simulink model "balance_car_measured_foc"  (R2025b)
settings: Solver=ode15s  StartTime=0.0  StopTime=6  MaxStep=0.00025  RelTol=1e-5  AbsTol=1e-7
PostLoadFcn:
  | addpath(fileparts(get_param(bdroot,'FileName')));addpath(fileparts(fileparts(get_param(bdroot,'FileName'))));p=balance_setup;addpath(fullfile(p.root,'模型','仿真模型','通用URDF','meshes'));
model workspace (MAT data in the model file):
  direction_convention = 'x_right_y_forward_v2'
  foc_config = [0.110387231165 2.4e-05 0.00887463966788 0.060318579 226.194672 5e-05 4 3 8.03 0.04 0.4 0.7 ... (31 elements, 1x31)]
  sensor_config = [1 0.314910266476 0.419379363666 0.000198810278564 0.000166561121409 0.00015843402401 0.005 44 0.0325 0.00147678407027 4.07299587781e-05 1.77121446999e-05 ... (342 elements, 1x342)]
  suite_config = [1 0.7 -0.00156420808869 0 0 0 0 0 0 0 0 0 ... (37 elements, 1x37)]
  terrain_dimensions = [0.3  0.120037494142  0.01; 0.3  0.1  0.01; 0.3  0.120037494142  0.01; 0.06  0.04  0.01]
  terrain_on = 0
  terrain_rotation_deg = [-1.43209618416; 0; 1.43209618416; 0]
  terrain_translation = [0  0.240124960956  -0.00349843823204; 0  0.35  -0.002; 0  0.459875039044  -0.00349843823204; -0.0662682  0.62  -0.0042]
values from neighbouring files (symbols this model uses):
  N = numel(t)    [screen_measured_pid.m]
  s = load(fullfile(folder,'simulation_measured.mat'),'o')    [analyze_course_odometry.m]    (also in build_measured_car.m = side{1}; diagnose_encoder_yaw_gate.m = jsondecode(fileread(fullfile(out,'summary.json'))); measured_car_reference.m = amplitude*(10*u^3-15*u^4+6*u^5); measured_ekf_step.m = [0 -v(3) v(2);v(3) 0 -v(1);-v(2) v(1) 0])
  Y = []    [identify_measured_foc.m]
undefined symbols (not defined in the file or in its folder): X, Z
libraries: sm_lib x48, nesl_utility x27
(part 2 of 2)

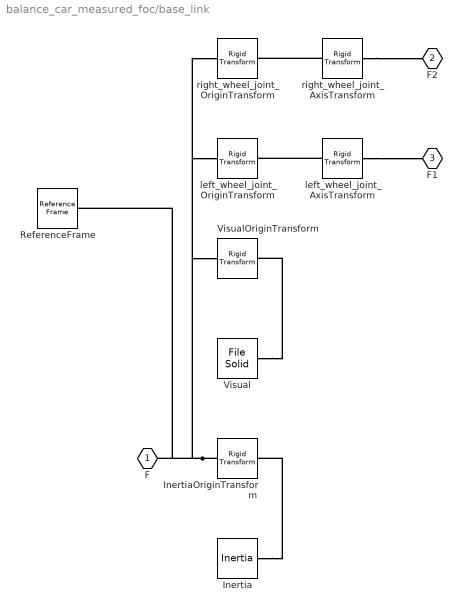
== system balance_car_measured_foc/base_link ==
  Inertia : sm_lib/Body Elements/Inertia  InertiaType=Custom  Mass=0.2771  MassUnits=kg  CenterOfMass=[0, 0, 0]  CenterOfMassUnits=m  MomentsOfInertia=[0.000311847668361045, 0.0006191390109428378, 0.000388176637385571]  MomentsOfInertiaUnits=kg*m^2  ProductsOfInertia=[3.850274462317628e-08, -1.767576624229698e-07, -2.823397326959528e-07]  ProductsOfInertiaUnits=kg*m^2  GraphicType=None  MarkerShape=Inertia  MarkerSize=20  GraphicVisPropType=SimpleVisualProperties  GraphicDiffuseColor=[0.5 0.5 0.5]  GraphicOpacity=1  GraphicSpecularColor=[0.5 0.5 0.5 1.0]  GraphicAmbientColor=[0.15 0.15 0.15 1.0]  GraphicEmissiveColor=[0.0 0.0 0.0 1.0]  GraphicShininess=75
  InertiaOriginTransform : sm_lib/Frames and Transforms/Rigid Transform  RotationMethod=RotationSequence  FollAlignAxisA=+X  BaseAlignAxisA=+Y  FollAlignAxisB=+Y  BaseAlignAxisB=+Z  RotationStandardAxis=+Z  RotationAngle=0  RotationAngleUnits=deg  RotationArbitraryAxis=[0 0 1]  RotationSequenceAxes=BaseAxes  RotationSequence=XYZ  RotationSequenceAngles=[0, 0, 0]  RotationSequenceAnglesUnits=rad  RotationMatrix=[1 0 0;0 1 0;0 0 1]  Quaternion=[1 0 0 0]  TranslationMethod=Cartesian  TranslationCartesianOffset=[-4.53146929236e-05, 5.71393596063e-05, 0.0365292274203]  TranslationCartesianOffsetUnits=m  TranslationStandardAxis=+Z  TranslationStandardOffset=0  TranslationStandardOffsetUnits=m  TranslationROffset=0  TranslationROffsetUnits=m  TranslationThetaOffset=0  TranslationThetaOffsetUnits=deg  TranslationZOffset=0  TranslationZOffsetUnits=m
  ReferenceFrame : sm_lib/Frames and Transforms/Reference Frame
  Visual : sm_lib/Body Elements/File Solid  ExtGeomFileName=body.stl  UnitType=Custom  ExtGeomFileUnits=m  StepReaderType=HEX  ExportConvexHullGeometry=off  InertiaType=Custom  BasedOnType=DensityFromFile  Density=1000  DensityUnits=kg/m^3  Mass=0  MassUnits=kg  CenterOfMass=[0, 0, 0]  CenterOfMassUnits=m  MomentsOfInertia=[0, 0, 0]  MomentsOfInertiaUnits=kg*m^2  ProductsOfInertia=[0, 0, 0]  ProductsOfInertiaUnits=kg*m^2  GraphicType=FromGeometry  MarkerShape=Sphere  MarkerSize=10  GraphicVisPropType=SimpleVisualProperties  GraphicDiffuseColor=[0.12, 0.4, 0.65]  GraphicOpacity=1  GraphicSpecularColor=[0.5 0.5 0.5 1.0]  GraphicAmbientColor=[0.15 0.15 0.15 1.0]  GraphicEmissiveColor=[0.0 0.0 0.0 1.0]  GraphicShininess=75  DoExposeReferenceFrame=on  SerializedFrames=<Frames/>
  VisualOriginTransform : sm_lib/Frames and Transforms/Rigid Transform  RotationMethod=RotationSequence  FollAlignAxisA=+X  BaseAlignAxisA=+Y  FollAlignAxisB=+Y  BaseAlignAxisB=+Z  RotationStandardAxis=+Z  RotationAngle=0  RotationAngleUnits=deg  RotationArbitraryAxis=[0 0 1]  RotationSequenceAxes=BaseAxes  RotationSequence=XYZ  RotationSequenceAngles=[0, 0, -1.570796326794897]  RotationSequenceAnglesUnits=rad  RotationMatrix=[1 0 0;0 1 0;0 0 1]  Quaternion=[1 0 0 0]  TranslationMethod=Cartesian  TranslationCartesianOffset=[0, 0, 0]  TranslationCartesianOffsetUnits=m  TranslationStandardAxis=+Z  TranslationStandardOffset=0  TranslationStandardOffsetUnits=m  TranslationROffset=0  TranslationROffsetUnits=m  TranslationThetaOffset=0  TranslationThetaOffsetUnits=deg  TranslationZOffset=0  TranslationZOffsetUnits=m
  left_wheel_joint_AxisTransform : sm_lib/Frames and Transforms/Rigid Transform  RotationMethod=ArbitraryAxis  FollAlignAxisA=+X  BaseAlignAxisA=+Y  FollAlignAxisB=+Y  BaseAlignAxisB=+Z  RotationStandardAxis=+Z  RotationAngle=1.570796326794897  RotationAngleUnits=rad  RotationArbitraryAxis=[-0, -1, 0]  RotationSequenceAxes=FollowerAxes  RotationSequence=XYX  RotationSequenceAngles=[0 0 0]  RotationSequenceAnglesUnits=deg  RotationMatrix=[1 0 0;0 1 0;0 0 1]  Quaternion=[1 0 0 0]  TranslationMethod=Cartesian  TranslationCartesianOffset=[0, 0, 0]  TranslationCartesianOffsetUnits=m  TranslationStandardAxis=+Z  TranslationStandardOffset=0  TranslationStandardOffsetUnits=m  TranslationROffset=0  TranslationROffsetUnits=m  TranslationThetaOffset=0  TranslationThetaOffsetUnits=deg  TranslationZOffset=0  TranslationZOffsetUnits=m
  left_wheel_joint_OriginTransform : sm_lib/Frames and Transforms/Rigid Transform  RotationMethod=RotationSequence  FollAlignAxisA=+X  BaseAlignAxisA=+Y  FollAlignAxisB=+Y  BaseAlignAxisB=+Z  RotationStandardAxis=+Z  RotationAngle=0  RotationAngleUnits=deg  RotationArbitraryAxis=[0 0 1]  RotationSequenceAxes=BaseAxes  RotationSequence=XYZ  RotationSequenceAngles=[0, 0, 0]  RotationSequenceAnglesUnits=rad  RotationMatrix=[1 0 0;0 1 0;0 0 1]  Quaternion=[1 0 0 0]  TranslationMethod=Cartesian  TranslationCartesianOffset=[-0.0662682, 0, 0]  TranslationCartesianOffsetUnits=m  TranslationStandardAxis=+Z  TranslationStandardOffset=0  TranslationStandardOffsetUnits=m  TranslationROffset=0  TranslationROffsetUnits=m  TranslationThetaOffset=0  TranslationThetaOffsetUnits=deg  TranslationZOffset=0  TranslationZOffsetUnits=m
  right_wheel_joint_AxisTransform : sm_lib/Frames and Transforms/Rigid Transform  RotationMethod=ArbitraryAxis  FollAlignAxisA=+X  BaseAlignAxisA=+Y  FollAlignAxisB=+Y  BaseAlignAxisB=+Z  RotationStandardAxis=+Z  RotationAngle=1.570796326794897  RotationAngleUnits=rad  RotationArbitraryAxis=[-0, -1, 0]  RotationSequenceAxes=FollowerAxes  RotationSequence=XYX  RotationSequenceAngles=[0 0 0]  RotationSequenceAnglesUnits=deg  RotationMatrix=[1 0 0;0 1 0;0 0 1]  Quaternion=[1 0 0 0]  TranslationMethod=Cartesian  TranslationCartesianOffset=[0, 0, 0]  TranslationCartesianOffsetUnits=m  TranslationStandardAxis=+Z  TranslationStandardOffset=0  TranslationStandardOffsetUnits=m  TranslationROffset=0  TranslationROffsetUnits=m  TranslationThetaOffset=0  TranslationThetaOffsetUnits=deg  TranslationZOffset=0  TranslationZOffsetUnits=m
  right_wheel_joint_OriginTransform : sm_lib/Frames and Transforms/Rigid Transform  RotationMethod=RotationSequence  FollAlignAxisA=+X  BaseAlignAxisA=+Y  FollAlignAxisB=+Y  BaseAlignAxisB=+Z  RotationStandardAxis=+Z  RotationAngle=0  RotationAngleUnits=deg  RotationArbitraryAxis=[0 0 1]  RotationSequenceAxes=BaseAxes  RotationSequence=XYZ  RotationSequenceAngles=[0, 0, 0]  RotationSequenceAnglesUnits=rad  RotationMatrix=[1 0 0;0 1 0;0 0 1]  Quaternion=[1 0 0 0]  TranslationMethod=Cartesian  TranslationCartesianOffset=[0.0662682, 0, 0]  TranslationCartesianOffsetUnits=m  TranslationStandardAxis=+Z  TranslationStandardOffset=0  TranslationStandardOffsetUnits=m  TranslationROffset=0  TranslationROffsetUnits=m  TranslationThetaOffset=0  TranslationThetaOffsetUnits=deg  TranslationZOffset=0  TranslationZOffsetUnits=m
  F : PMIOPort  Side=Left
  F2 : PMIOPort  Port=2  Side=Right
  F1 : PMIOPort  Port=3  Side=Right
  connections:
  Inertia/RConn1 -- InertiaOriginTransform/RConn1
  ReferenceFrame/RConn1 -- InertiaOriginTransform/LConn1 -- VisualOriginTransform/LConn1 -- left_wheel_joint_OriginTransform/LConn1 -- right_wheel_joint_OriginTransform/LConn1 -- F/RConn1
  Visual/RConn1 -- VisualOriginTransform/RConn1
  left_wheel_joint_AxisTransform/RConn1 -- F1/RConn1
  left_wheel_joint_AxisTransform/LConn1 -- left_wheel_joint_OriginTransform/RConn1
  right_wheel_joint_AxisTransform/RConn1 -- F2/RConn1
  right_wheel_joint_AxisTransform/LConn1 -- right_wheel_joint_OriginTransform/RConn1

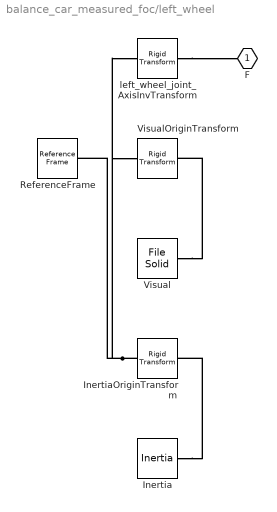
== system balance_car_measured_foc/left_wheel ==
  Inertia : sm_lib/Body Elements/Inertia  InertiaType=Custom  Mass=0.06270000000000001  MassUnits=kg  CenterOfMass=[0, 0, 0]  CenterOfMassUnits=m  MomentsOfInertia=[2.996788998409583e-05, 1.917831991019923e-05, 1.917831830082714e-05]  MomentsOfInertiaUnits=kg*m^2  ProductsOfInertia=[-7.252640957165455e-12, -1.265848447928984e-12, -3.833693155565584e-12]  ProductsOfInertiaUnits=kg*m^2  GraphicType=None  MarkerShape=Inertia  MarkerSize=20  GraphicVisPropType=SimpleVisualProperties  GraphicDiffuseColor=[0.5 0.5 0.5]  GraphicOpacity=1  GraphicSpecularColor=[0.5 0.5 0.5 1.0]  GraphicAmbientColor=[0.15 0.15 0.15 1.0]  GraphicEmissiveColor=[0.0 0.0 0.0 1.0]  GraphicShininess=75
  InertiaOriginTransform : sm_lib/Frames and Transforms/Rigid Transform  RotationMethod=RotationSequence  FollAlignAxisA=+X  BaseAlignAxisA=+Y  FollAlignAxisB=+Y  BaseAlignAxisB=+Z  RotationStandardAxis=+Z  RotationAngle=0  RotationAngleUnits=deg  RotationArbitraryAxis=[0 0 1]  RotationSequenceAxes=BaseAxes  RotationSequence=XYZ  RotationSequenceAngles=[0, 0, 0]  RotationSequenceAnglesUnits=rad  RotationMatrix=[1 0 0;0 1 0;0 0 1]  Quaternion=[1 0 0 0]  TranslationMethod=Cartesian  TranslationCartesianOffset=[0.00137780420767, 3.60871449808e-09, -5.37617755869e-09]  TranslationCartesianOffsetUnits=m  TranslationStandardAxis=+Z  TranslationStandardOffset=0  TranslationStandardOffsetUnits=m  TranslationROffset=0  TranslationROffsetUnits=m  TranslationThetaOffset=0  TranslationThetaOffsetUnits=deg  TranslationZOffset=0  TranslationZOffsetUnits=m
  ReferenceFrame : sm_lib/Frames and Transforms/Reference Frame
  Visual : sm_lib/Body Elements/File Solid  ExtGeomFileName=right_wheel.stl  UnitType=Custom  ExtGeomFileUnits=m  StepReaderType=HEX  ExportConvexHullGeometry=off  InertiaType=Custom  BasedOnType=DensityFromFile  Density=1000  DensityUnits=kg/m^3  Mass=0  MassUnits=kg  CenterOfMass=[0, 0, 0]  CenterOfMassUnits=m  MomentsOfInertia=[0, 0, 0]  MomentsOfInertiaUnits=kg*m^2  ProductsOfInertia=[0, 0, 0]  ProductsOfInertiaUnits=kg*m^2  GraphicType=FromGeometry  MarkerShape=Sphere  MarkerSize=10  GraphicVisPropType=SimpleVisualProperties  GraphicDiffuseColor=[0.16, 0.18, 0.16]  GraphicOpacity=1  GraphicSpecularColor=[0.5 0.5 0.5 1.0]  GraphicAmbientColor=[0.15 0.15 0.15 1.0]  GraphicEmissiveColor=[0.0 0.0 0.0 1.0]  GraphicShininess=75  DoExposeReferenceFrame=on  SerializedFrames=<Frames/>
  VisualOriginTransform : sm_lib/Frames and Transforms/Rigid Transform  RotationMethod=RotationSequence  FollAlignAxisA=+X  BaseAlignAxisA=+Y  FollAlignAxisB=+Y  BaseAlignAxisB=+Z  RotationStandardAxis=+Z  RotationAngle=0  RotationAngleUnits=deg  RotationArbitraryAxis=[0 0 1]  RotationSequenceAxes=BaseAxes  RotationSequence=XYZ  RotationSequenceAngles=[0, 0, -1.570796326794897]  RotationSequenceAnglesUnits=rad  RotationMatrix=[1 0 0;0 1 0;0 0 1]  Quaternion=[1 0 0 0]  TranslationMethod=Cartesian  TranslationCartesianOffset=[0, 0, 0]  TranslationCartesianOffsetUnits=m  TranslationStandardAxis=+Z  TranslationStandardOffset=0  TranslationStandardOffsetUnits=m  TranslationROffset=0  TranslationROffsetUnits=m  TranslationThetaOffset=0  TranslationThetaOffsetUnits=deg  TranslationZOffset=0  TranslationZOffsetUnits=m
  left_wheel_joint_AxisInvTransform : sm_lib/Frames and Transforms/Rigid Transform  RotationMethod=ArbitraryAxis  FollAlignAxisA=+X  BaseAlignAxisA=+Y  FollAlignAxisB=+Y  BaseAlignAxisB=+Z  RotationStandardAxis=+Z  RotationAngle=1.570796326794897  RotationAngleUnits=rad  RotationArbitraryAxis=[-0, -1, 0]  RotationSequenceAxes=FollowerAxes  RotationSequence=XYX  RotationSequenceAngles=[0 0 0]  RotationSequenceAnglesUnits=deg  RotationMatrix=[1 0 0;0 1 0;0 0 1]  Quaternion=[1 0 0 0]  TranslationMethod=Cartesian  TranslationCartesianOffset=[0, 0, 0]  TranslationCartesianOffsetUnits=m  TranslationStandardAxis=+Z  TranslationStandardOffset=0  TranslationStandardOffsetUnits=m  TranslationROffset=0  TranslationROffsetUnits=m  TranslationThetaOffset=0  TranslationThetaOffsetUnits=deg  TranslationZOffset=0  TranslationZOffsetUnits=m
  F : PMIOPort  Side=Left
  connections:
  Inertia/RConn1 -- InertiaOriginTransform/RConn1
  ReferenceFrame/RConn1 -- InertiaOriginTransform/LConn1 -- VisualOriginTransform/LConn1 -- left_wheel_joint_AxisInvTransform/LConn1
  Visual/RConn1 -- VisualOriginTransform/RConn1
  left_wheel_joint_AxisInvTransform/RConn1 -- F/RConn1

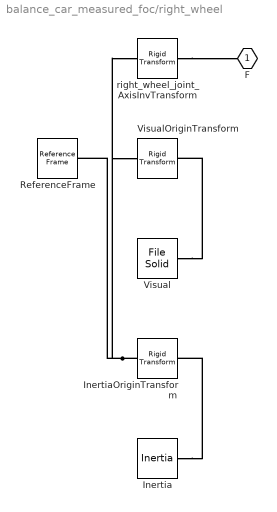
== system balance_car_measured_foc/right_wheel ==
  Inertia : sm_lib/Body Elements/Inertia  InertiaType=Custom  Mass=0.06270000000000001  MassUnits=kg  CenterOfMass=[0, 0, 0]  CenterOfMassUnits=m  MomentsOfInertia=[2.996788998409583e-05, 1.917831991019924e-05, 1.917831830082714e-05]  MomentsOfInertiaUnits=kg*m^2  ProductsOfInertia=[7.252640958073256e-12, 1.265848450812081e-12, -3.83369315636605e-12]  ProductsOfInertiaUnits=kg*m^2  GraphicType=None  MarkerShape=Inertia  MarkerSize=20  GraphicVisPropType=SimpleVisualProperties  GraphicDiffuseColor=[0.5 0.5 0.5]  GraphicOpacity=1  GraphicSpecularColor=[0.5 0.5 0.5 1.0]  GraphicAmbientColor=[0.15 0.15 0.15 1.0]  GraphicEmissiveColor=[0.0 0.0 0.0 1.0]  GraphicShininess=75
  InertiaOriginTransform : sm_lib/Frames and Transforms/Rigid Transform  RotationMethod=RotationSequence  FollAlignAxisA=+X  BaseAlignAxisA=+Y  FollAlignAxisB=+Y  BaseAlignAxisB=+Z  RotationStandardAxis=+Z  RotationAngle=0  RotationAngleUnits=deg  RotationArbitraryAxis=[0 0 1]  RotationSequenceAxes=BaseAxes  RotationSequence=XYZ  RotationSequenceAngles=[0, 0, 0]  RotationSequenceAnglesUnits=rad  RotationMatrix=[1 0 0;0 1 0;0 0 1]  Quaternion=[1 0 0 0]  TranslationMethod=Cartesian  TranslationCartesianOffset=[-0.00137780420767, -3.60871449673e-09, -5.37617755869e-09]  TranslationCartesianOffsetUnits=m  TranslationStandardAxis=+Z  TranslationStandardOffset=0  TranslationStandardOffsetUnits=m  TranslationROffset=0  TranslationROffsetUnits=m  TranslationThetaOffset=0  TranslationThetaOffsetUnits=deg  TranslationZOffset=0  TranslationZOffsetUnits=m
  ReferenceFrame : sm_lib/Frames and Transforms/Reference Frame
  Visual : sm_lib/Body Elements/File Solid  ExtGeomFileName=left_wheel.stl  UnitType=Custom  ExtGeomFileUnits=m  StepReaderType=HEX  ExportConvexHullGeometry=off  InertiaType=Custom  BasedOnType=DensityFromFile  Density=1000  DensityUnits=kg/m^3  Mass=0  MassUnits=kg  CenterOfMass=[0, 0, 0]  CenterOfMassUnits=m  MomentsOfInertia=[0, 0, 0]  MomentsOfInertiaUnits=kg*m^2  ProductsOfInertia=[0, 0, 0]  ProductsOfInertiaUnits=kg*m^2  GraphicType=FromGeometry  MarkerShape=Sphere  MarkerSize=10  GraphicVisPropType=SimpleVisualProperties  GraphicDiffuseColor=[0.16, 0.18, 0.16]  GraphicOpacity=1  GraphicSpecularColor=[0.5 0.5 0.5 1.0]  GraphicAmbientColor=[0.15 0.15 0.15 1.0]  GraphicEmissiveColor=[0.0 0.0 0.0 1.0]  GraphicShininess=75  DoExposeReferenceFrame=on  SerializedFrames=<Frames/>
  VisualOriginTransform : sm_lib/Frames and Transforms/Rigid Transform  RotationMethod=RotationSequence  FollAlignAxisA=+X  BaseAlignAxisA=+Y  FollAlignAxisB=+Y  BaseAlignAxisB=+Z  RotationStandardAxis=+Z  RotationAngle=0  RotationAngleUnits=deg  RotationArbitraryAxis=[0 0 1]  RotationSequenceAxes=BaseAxes  RotationSequence=XYZ  RotationSequenceAngles=[0, 0, -1.570796326794897]  RotationSequenceAnglesUnits=rad  RotationMatrix=[1 0 0;0 1 0;0 0 1]  Quaternion=[1 0 0 0]  TranslationMethod=Cartesian  TranslationCartesianOffset=[0, 0, 0]  TranslationCartesianOffsetUnits=m  TranslationStandardAxis=+Z  TranslationStandardOffset=0  TranslationStandardOffsetUnits=m  TranslationROffset=0  TranslationROffsetUnits=m  TranslationThetaOffset=0  TranslationThetaOffsetUnits=deg  TranslationZOffset=0  TranslationZOffsetUnits=m
  right_wheel_joint_AxisInvTransform : sm_lib/Frames and Transforms/Rigid Transform  RotationMethod=ArbitraryAxis  FollAlignAxisA=+X  BaseAlignAxisA=+Y  FollAlignAxisB=+Y  BaseAlignAxisB=+Z  RotationStandardAxis=+Z  RotationAngle=1.570796326794897  RotationAngleUnits=rad  RotationArbitraryAxis=[-0, -1, 0]  RotationSequenceAxes=FollowerAxes  RotationSequence=XYX  RotationSequenceAngles=[0 0 0]  RotationSequenceAnglesUnits=deg  RotationMatrix=[1 0 0;0 1 0;0 0 1]  Quaternion=[1 0 0 0]  TranslationMethod=Cartesian  TranslationCartesianOffset=[0, 0, 0]  TranslationCartesianOffsetUnits=m  TranslationStandardAxis=+Z  TranslationStandardOffset=0  TranslationStandardOffsetUnits=m  TranslationROffset=0  TranslationROffsetUnits=m  TranslationThetaOffset=0  TranslationThetaOffsetUnits=deg  TranslationZOffset=0  TranslationZOffsetUnits=m
  F : PMIOPort  Side=Left
  connections:
  Inertia/RConn1 -- InertiaOriginTransform/RConn1
  ReferenceFrame/RConn1 -- InertiaOriginTransform/LConn1 -- VisualOriginTransform/LConn1 -- right_wheel_joint_AxisInvTransform/LConn1
  Visual/RConn1 -- VisualOriginTransform/RConn1
  right_wheel_joint_AxisInvTransform/RConn1 -- F/RConn1

== matlab function balance_car_measured_foc/Measured_FOC ==
  data: mechanics input; out output; iq input; t input; cfg input
function out=measured_vehicle_actuator(mechanics,iq,t,cfg)
%#codegen
% Mechanics are supplied by Multibody. Do not integrate wheel inertia here.
persistent x
if isempty(x),x=measured_foc_initial(mechanics(1:2));end
q=mechanics(1:2);w=mechanics(3:4);refs=[0 0;iq(1) iq(2)];tick=round(t/cfg(6));torque=zeros(2,1);steps=round(cfg(31));y=zeros(14,2);
for k=0:steps-1
 [x,y]=measured_foc_step(x,refs,q+w*(k*cfg(6)),w,tick+k,cfg);torque=torque+y(1,:)';
end
friction=[cfg(17);cfg(18)].*w+[cfg(19);cfg(20)].*tanh(w/.5);
out=[torque/steps-friction;y(:)];
end

== matlab function balance_car_measured_foc/Balance_Controller ==
  data: raw input; out output; cfg input
function out=balance_suite_controller(raw,cfg)
%#codegen
% raw=[time x vx y vy z vz qw qx qy qz wx wy wz]，角速度在世界坐标。
% out=[实际tau(2) state(6) ref(6) force(3) torque(3) fall 执行指令(2) PID目标(2)]。
% cfg(16)=2时执行指令是iq/A；其余模式为转矩/Nm。
% 外部XYZ为右/前/上；内部控制坐标仍用前/左/上，保留已整定增益。
raw=[raw(1);raw(4);raw(5);-raw(2);-raw(3);raw(6);raw(7); ...
 raw(8);raw(10);-raw(9);raw(11);raw(13);-raw(12);raw(14)];
persistent distance prevV velocityIntegral pitchIntegral yawIntegral
if isempty(distance)
 distance=0;prevV=0;velocityIntegral=0;pitchIntegral=0;yawIntegral=0;
end
t=raw(1); qw=raw(8);qx=raw(9);qy=raw(10);qz=raw(11);
R=[1-2*(qy^2+qz^2) 2*(qx*qy-qw*qz) 2*(qx*qz+qw*qy); ...
   2*(qx*qy+qw*qz) 1-2*(qx^2+qz^2) 2*(qy*qz-qw*qx); ...
   2*(qx*qz-qw*qy) 2*(qy*qz+qw*qx) 1-2*(qx^2+qy^2)];
pitch=atan2(-R(3,1),hypot(R(1,1),R(2,1)));yaw=atan2(R(2,1),R(1,1));
roll=atan2(R(3,2),R(3,3)); wb=R'*raw(12:14);
pitchRate=cos(roll)*wb(2)-sin(roll)*wb(3);
yawRate=(sin(roll)*wb(2)+cos(roll)*wb(3))/cos(pitch);
v=cos(yaw)*raw(3)+sin(yaw)*raw(5);
Ts=cfg(31);
if t>0,distance=distance+Ts*(prevV+v)/2;end
prevV=v;
state=[distance;v;pitch-cfg(3);pitchRate;yaw;yawRate];
ref=zeros(6,1);F=zeros(3,1);T=zeros(3,1);scenario=round(cfg(1));
fast=round(cfg(34))==1;
if scenario==2 % 指令行驶：0.3m前进，随后后退到0.1m。
 if fast
  [p1,v1]=smoothmove(t,1,1.2,.30);[p2,v2]=smoothmove(t,3.8,1.2,-.20);
 else
  [p1,v1]=smoothmove(t,1,3,.30);[p2,v2]=smoothmove(t,6,2,-.20);
 end
 ref(1)=p1+p2;ref(2)=v1+v2;
elseif scenario==3 % 原地转60°，随后返回20°。
 if fast
  [a,w]=smoothmove(t,1,1.2,pi/3);[a2,w2]=smoothmove(t,4,1.2,-2*pi/9);
 else
  [a,w]=smoothmove(t,1,2,pi/3);[a2,w2]=smoothmove(t,5,2,-2*pi/9);
 end
 ref(5)=a+a2;ref(6)=w+w2;
elseif scenario==4 % 向前运动同时转弯。
 if fast
  [s,vs]=smoothmove(t,1,3,.6);[a,w]=smoothmove(t,1.5,1.5,pi/3);
 else
  [s,vs]=smoothmove(t,1,6,.6);[a,w]=smoothmove(t,2,3,pi/3);
 end
 ref(1)=s;ref(2)=vs;ref(5)=a;ref(6)=w;
elseif scenario==5 % 轮轴处的外力及绕竖直轴的外转矩脉冲。
 if t>=2 && t<2.15,F(1)=.4;end
 if t>=4 && t<4.15,T(3)=.002;end
elseif scenario==6 % 地形路线：经过缓坡、平台、下坡和单侧小凸起。
 [s,vs]=smoothmove(t,1,8,.75);ref(1)=s;ref(2)=vs;
elseif scenario==7 % 恒定扰动：比较两种控制器的稳态误差。
 if t>=2,F(1)=.08;T(3)=.0004;end
elseif scenario==8 % 明显坡道：上坡、平台、下坡、单侧凸起。
 [s,vs]=smoothmove(t,1,20,cfg(36));ref(1)=s;ref(2)=vs;
elseif scenario==9 % 斜面中段停12秒，随后继续通过坡顶与下坡。
 [s1,v1]=smoothmove(t,1,6,cfg(35));
 [s2,v2]=smoothmove(t,19,11,cfg(36)-cfg(35));
 ref(1)=s1+s2;ref(2)=v1+v2;
end
error=state-ref;
pidTarget=zeros(2,1);
if cfg(16)<.5
 K=reshape(cfg(4:15),2,6);effort=-K*error;
else
 targetV=clamp(ref(2)+cfg(22)*(ref(1)-state(1)),cfg(23));
 velocityError=targetV-v;
 vi=clamp(velocityIntegral+Ts*velocityError,cfg(25));
 targetUnclamped=cfg(20)*velocityError+cfg(21)*vi;
 targetPitch=clamp(targetUnclamped,cfg(24));
 pitchError=state(3)-targetPitch;
 piCandidate=clamp(pitchIntegral+Ts*pitchError,cfg(26));
 yawError=atan2(sin(ref(5)-yaw),cos(ref(5)-yaw));
 yi=clamp(yawIntegral+Ts*yawError,cfg(30));
 effort=[cfg(17)*pitchError+cfg(18)*piCandidate+cfg(19)*pitchRate; ...
  cfg(27)*yawError+cfg(28)*yi+cfg(29)*(ref(6)-yawRate)];
 % 转矩或倾角饱和时冻结相关积分。
 if max(abs([(effort(1)-effort(2))/2;(effort(1)+effort(2))/2]))<=cfg(2)
  pitchIntegral=piCandidate;yawIntegral=yi;
  if abs(targetUnclamped)<=cfg(24),velocityIntegral=vi;end
 end
 pidTarget=[targetV;targetPitch];
end
% effort(1)=左右转矩和，effort(2)=右减左。
tau=[(effort(1)-effort(2))/2;(effort(1)+effort(2))/2];
limit=cfg(2);
command=max(-limit,min(limit,tau));
tau=command.*[cfg(32);cfg(33)]; % 显式列向量，避免Simulink向量方向推断差异
if cfg(16)>1.5
 tau=tau*cfg(37); % 理想电流跟踪；实际Kt=标称Kt×左右执行增益。
end
% 外力/外转矩转换回实际世界XYZ（右/前/上）。
F=[-F(2);F(1);F(3)];T=[-T(2);T(1);T(3)];
out=[tau;state;ref;F;T;double(abs(pitch)>pi/4 || abs(roll)>pi/6);command;pidTarget];
end

function y=clamp(x,limit)
y=max(-limit,min(limit,x));
end

function [p,v]=smoothmove(t,start,duration,amplitude)
u=max(0,min(1,(t-start)/duration));
p=amplitude*(10*u^3-15*u^4+6*u^5);
if t<=start || t>=start+duration,v=0;
else,v=amplitude*(30*u^2-60*u^3+30*u^4)/duration;end
end

== matlab function balance_car_measured_foc/Measured_sensors ==
  data: raw input; sensed output; actuator input; cfg input
function sensed=measured_vehicle_sensors(raw,actuator,cfg)
%#codegen
% Reproduce MPU scaling, approximate hardware bandwidth and original complementary filter.
% raw world frame: X right, Y forward, Z up. Encoder observations come from 5kHz actuator.
persistent prevV accLP gyroLP accNoise gyroNoise angles seed historyAcc historyGyro
sensed=raw;
q=raw(8:11);R=rotation(q);dt=cfg(7);v=[raw(3);raw(5);raw(7)];
if isempty(prevV)
 prevV=v;accLP=R'*[0;0;1];gyroLP=R'*raw(12:14);accNoise=zeros(3,1);gyroNoise=zeros(3,1);angles=zeros(3,1);seed=9259;
 angles(1)=atan2(accLP(2),accLP(3));angles(2)=atan2(-accLP(1),hypot(accLP(2),accLP(3)));angles(3)=atan2(-R(1,2),R(2,2));
 historyAcc=zeros(12,3,3);historyGyro=zeros(12,3,3);
end
if cfg(1)<.5,prevV=v;return;end
accel=(v-prevV)/dt;prevV=v;acc=R'*([0;0;9.80665]+accel)/9.80665;gyro=R'*raw(12:14);
a=dt/(1/(2*pi*cfg(8))+dt);accLP=accLP+a*(acc-accLP);gyroLP=gyroLP+a*(gyro-gyroLP);
z=zeros(6,1);
for k=1:3
 seed=mod(1664525*seed+1013904223,4294967296);u=(seed+1)/4294967297;
 seed=mod(1664525*seed+1013904223,4294967296);vnoise=(seed+1)/4294967297;r=sqrt(-2*log(u));z(2*k-1)=r*cos(2*pi*vnoise);z(2*k)=r*sin(2*pi*vnoise);
end
speed=.5*(abs(actuator(15))+abs(actuator(29)));u=min(speed/10,2);
bankA=zeros(3,3);bankG=zeros(3,3);
for j=1:3
 base=73+45*(j-1);A=reshape(cfg(base:base+35),12,3);L=reshape(cfg(base+36:base+44),3,3);
 bankA(:,j)=-sum(A.*historyAcc(:,:,j),1)'+L*z(1:3);historyAcc(2:12,:,j)=historyAcc(1:11,:,j);historyAcc(1,:,j)=bankA(:,j)';
 base=73+45*(j+2);A=reshape(cfg(base:base+35),12,3);L=reshape(cfg(base+36:base+44),3,3);
 bankG(:,j)=-sum(A.*historyGyro(:,:,j),1)'+L*z(4:6);historyGyro(2:12,:,j)=historyGyro(1:11,:,j);historyGyro(1,:,j)=bankG(:,j)';
end
weights=[max(1-u,0);1-max(1-u,0)-max(u-1,0);max(u-1,0)];accNoise=bankA*weights;gyroNoise=bankG*weights;
acc=round(max(-2,min(2,cfg(72)*accLP+accNoise))*16384)/16384;
gyro=gyroLP+[cfg(4);cfg(5);cfg(6)]+gyroNoise;gyro=round(max(-500*pi/180,min(500*pi/180,gyro))*65.5*180/pi)/(65.5*180/pi);
ap=atan2(acc(2),acc(3));ar=atan2(-acc(1),hypot(acc(2),acc(3)));
angles(1)=.98*(angles(1)+gyro(1)*dt)+.02*ap;angles(2)=.98*(angles(2)+gyro(2)*dt)+.02*ar;angles(3)=angles(3)+gyro(3)*dt;
cx=cos(angles(1)/2);sx=sin(angles(1)/2);cy=cos(angles(2)/2);sy=sin(angles(2)/2);cz=cos(angles(3)/2);sz=sin(angles(3)/2);
quat=[cx*cy*cz+sx*sy*sz;sx*cy*cz-cx*sy*sz;cx*sy*cz+sx*cy*sz;cx*cy*sz-sx*sy*cz];
sensed(8:11)=quat;Rs=rotation(quat);sensed(12:14)=Rs*gyro;
forward=cfg(9)*(.5*(actuator(15)+actuator(29))-gyro(1));
sensed(3)=-sin(angles(3))*forward;sensed(5)=cos(angles(3))*forward;
end
function R=rotation(q)
w=q(1);x=q(2);y=q(3);z=q(4);R=[1-2*(y*y+z*z) 2*(x*y-w*z) 2*(x*z+w*y);2*(x*y+w*z) 1-2*(x*x+z*z) 2*(y*z-w*x);2*(x*z-w*y) 2*(y*z+w*x) 1-2*(x*x+y*y)];
end

== matlab function balance_car_measured_foc/Actual_control_log ==
  data: c input; y output; tau input
function y=combine(c,tau)
%#codegen
y=[tau;c(3:25)];
end
